simulink model "ASM_AnimationInterface"  (R2024a)
settings: Solver=ode1  StartTime=SIM.tstart.v  StopTime=SIM.tend.v  FixedStep=SIM.StepSize.v  RelTol=1e-3
PostLoadFcn:
  | , if any(exist('dsrtsu_mdlpostloadfcn', 'file') ~= 0), dsrtsu_mdlpostloadfcn('Execute', bdroot); end,
undefined symbols (not defined in the file): a0b2, b98103fe8ad365046cd0, dsmsi, MDL, SIM
libraries: simulink x22, dsmsilib x15, dsmpblib x4, ASM_Environment_lib x1
(part 1 of 7)
settings Model: RTICANMMDATA=struct('GeneralSetupData',struct('modelroot','C:\_GIT\ASM\Demo\Common\Simulation\Models','generalsettings',struct('filesettings',struct('destfolder',struct('Name','RTICANMM_FILES','Check',1),'buildfolder',struct('Name','.','Check',1),'AbsDestfolder',struct('Name','C:\_GIT\ASM\Demo\Common\Simulation\Models\RTICANMM_FILES'),'AbsBuildfolder',struct('Name','C:\_GIT\ASM\Demo\Common\Simulation\Models'))),'options',struct('addpaths',1,'rmpaths',1,'addtrcexclusion',true,'cannavigator',struct('checkmonitoring',0),'show_usrtrc',0,'use_usrtrc',0),'advanced',struct('options',ones(1,100)),'MPSetup',{{}},'RTI',struct('Type','GRT','Ver','','Date',''),'modelname','ASM_AnimationInterface','block','ASM_AnimationInterface'))  RTILINMMDATA=struct('GeneralSetupData',[])  DSRTSU_INTERNAL_RTI_VER=680  DSRTSU_INTERNAL_RTI_TYPE=rti1202  DSRTSU_INTERNAL_MDBS_VER=10  DSRTSU_INTERNAL_RTIFPGA=231  DSMPB_ID_DATA={'213406',struct('BlockId','196758cd-f01c-424e-aa71-f09de9b2c735','SignalIds',{{'6bbc41e1-0e49-4599-bed1-e27503c69a6b','b0969e61-917d-4221-8d62-1269ab223ac8'}}),'213407',struct('BlockId','6fc9ca26-9143-4720-acd9-f350a67d1c14','SignalIds',{{'88eab67c-f0eb-465f-8586-3b7bd00cb24a'}}),'213408',struct('BlockId','3cf7e26e-2ba5-4f6c-9896-28141b6d82c0','SignalIds',{{'8521c402-61b4-4fd4-94cf-d9926b9aa0e5'}}),'213409',struct('BlockId','5820cfdf-8ef4-4d35-adbb-082004934516','SignalIds',{{'6ca39ae5-80bb-46c1-91c4-90194903fd58','bdebb698-3ad2-4907-af9b-3ee7a1752205'}})}  DSRTSU_INTERNAL_RTISTBM_VER=26.1  Creator=RainerF  LastModifiedBy=dSPACE GmbH
settings SolverCC: AlgebraicLoopSolver=TrustRegion
settings DataIOCC: LimitDataPoints=on  SaveFormat=Structure  SignalLoggingSaveFormat=ModelDataLogs  SaveOutput=off  SignalLogging=off  DSMLogging=off  SaveTime=off  ReturnWorkspaceOutputs=off  SignalLoggingName=sigsOut
settings OptimizationCC: BlockReduction=off  BooleanDataType=off  ConditionallyExecuteInputs=off  OptimizeBlockIOStorage=off  BufferReuse=off  ReuseModelBlockBuffer=off  GlobalBufferReuse=off  ExpressionFolding=off  ExpressionDepthLimit=2147483647  LocalBlockOutputs=off  InitFltsAndDblsToZero=on  LifeSpan=inf  OptimizeDataStoreBuffers=off  BusAssignmentInplaceUpdate=off
settings DebuggingCC: SignalInfNanChecking=warning  SaveWithParameterizedLinksMsg=none  SignalResolutionControl=TryResolveAllWithWarning  MultiTaskDSMMsg=warning  MultiTaskCondExecSysMsg=none  CheckMatrixSingularityMsg=warning  FcnCallInpInsideContextMsg=warning  UnconnectedInputMsg=warning  UnconnectedOutputMsg=warning  UnconnectedLineMsg=warning  AllowSymbolicDim=off  StateNameClashWarn=warning  PregeneratedLibrarySubsystemCodeDiagnostic=none  StrictBusMsg=ErrorOnBusTreatedAsVector  NonBusSignalsTreatedAsBus=error  SFUnexpectedBacktrackingDiag=warning  SFNoUnconditionalDefaultTransitionDiag=warning  SFExecutionAtInitializationDiag=none  ArithmeticOperatorsInVariantConditions=warning
settings HardwareCC: ProdBitPerPointer=32  ProdBitPerSizeT=32  ProdBitPerPtrDiffT=32  ProdLargestAtomicFloat=None  ProdWordSize=32  ProdLongLongMode=on  ProdHWDeviceType=Specified  TargetIntDivRoundTo=Zero  TargetEndianess=LittleEndian
settings ModelReferenceCC: EnableRefExpFcnMdlSchedulingChecks=on  PropagateSignalLabelsOutOfModel=off
settings SFSimCC: SimUseLocalCustomCode=off  CustomCodeUndefinedFunction=UseInterfaceOnly
settings RTWCC: Description=dSPACE DS1006 Hardware Platform  RetainRTWFile=on  RTWUseLocalCustomCode=off  GPUComputeCapability=3.5  DLArmComputeVersion=19.05
settings CodeAppCC: StateflowObjectComments=on
settings GRTTargetCC: TargetFcnLib=ansi_tfl_tmw.mat  TargetLangStandard=C89/C90 (ANSI)  CombineOutputUpdateFcns=off  GRTInterface=on
settings ConfigComp: CovMetricSettings=dw  CovSaveCumulativeToWorkspaceVar=on  CovSaveSingleToWorkspaceVar=on  CovExternalEMLEnable=off  CovSFcnEnable=off

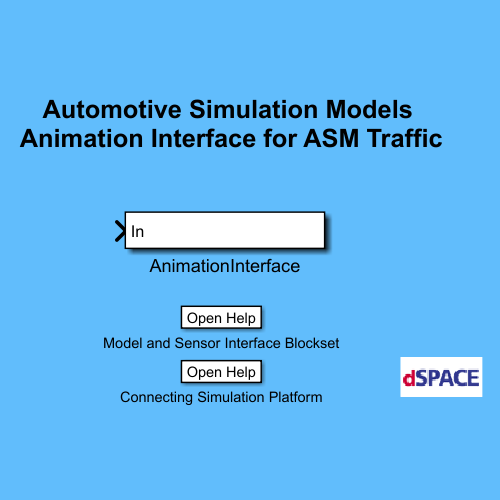
[thumbnail: Simulink's stored preview of the top-level diagram]
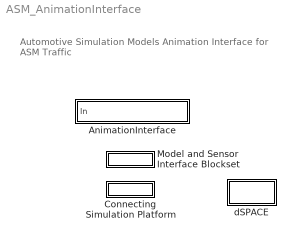
== system ASM_AnimationInterface ==
  note: Automotive Simulation Models
      | Animation Interface for ASM Traffic
  AnimationInterface : Subsystem  Tag=AnimationInterface
  Connecting Simulation Platform : Subsystem
      settings: OpenFcn=dsmsi_help('Help_ConnectingSimulationPlatforms')
      mask Display: disp('Open Help');
  Model and Sensor Interface Blockset : Subsystem
      settings: OpenFcn=dsmsi_help('HELP')
      mask Display: disp('Open Help');
  dSPACE : Subsystem
      mask Display: image(imread('asm_lib_dslogo.tif'));

== system ASM_AnimationInterface/AnimationInterface ==
  note: Animation Interface
  In : Inport
  ANIMATION_INTERFACE : Subsystem
  Bus Selector : BusSelector  OutputSignals=Environment.Animation.Sw_AnimationInterface[0Disabled|1Enabled],Environment.Animation.ManeuverState[]
  DriverAssistance_Animation : BusSelector  OutputSignals=DomainControl.DriverAssistance.Animation  OutputAsBus=on
  Drivetrain_Animation : BusSelector  OutputSignals=Drivetrain.Animation  OutputAsBus=on
  Environment_Animation : BusSelector  OutputSignals=Environment.Animation  OutputAsBus=on
  FcnCall : Subsystem
  Fellow_Doors : Subsystem
  Fellow_Lights : Subsystem
  OpenAnimationInterfaceModel : Subsystem
      settings: OpenFcn=|
      | InterfaceModel = 'ASM_AnimationInterface';
      | 
      | try
      |     open_system(InterfaceModel);                         catch
      |     errordlg(['ERROR opening Animation interface: ',InterfaceModel,'.slx']);
      | end
      mask Display: disp('Open ASM_AnimationInterface')
  Rate Transition{,1..3} (4 alike) : RateTransition  Integrity=off  OutPortSampleTimeOpt=Inherit
  VehicleDynamics_Animation : BusSelector  OutputSignals=VehicleDynamics.Animation  OutputAsBus=on
  Vehicle_Doors : Subsystem
  Vehicle_Lights : Subsystem
  wires:
  In/1 -> Bus Selector/1, DriverAssistance_Animation/1, Drivetrain_Animation/1, Environment_Animation/1, VehicleDynamics_Animation/1
  VehicleDynamics_Animation/1 -> Rate Transition3/1
  DriverAssistance_Animation/1 -> Rate Transition/1
  Environment_Animation/1 -> Rate Transition2/1
  Rate Transition/1 -> ANIMATION_INTERFACE/1(DriverAssistance_Animation)
  Rate Transition1/1 -> ANIMATION_INTERFACE/2(Drivetrain_Animation)
  Drivetrain_Animation/1 -> Rate Transition1/1
  Bus Selector/2 -> FcnCall/1(ManeuverState[])  "<ManeuverState[]>"
  FcnCall/1(FcnCallEvent[]) -> ANIMATION_INTERFACE/Trigger
  Rate Transition3/1 -> Vehicle_Lights/1(VehicleDynamics_Animation), ANIMATION_INTERFACE/3(VehicleDynamics_Animation)
  Fellow_Lights/1(Fellow_Light) -> ANIMATION_INTERFACE/6(Fellow_Lights)
  Vehicle_Lights/1(ASM_Vehicle_Lights) -> ANIMATION_INTERFACE/5(ASM_Vehicle_Lights)
  Rate Transition2/1 -> Fellow_Lights/1(Environment_Animation), Vehicle_Doors/1(Environment_Animation), Fellow_Doors/1(Environment_Animation), Vehicle_Lights/2(Environment_Animation), ANIMATION_INTERFACE/4(Environment_Animation)
  Vehicle_Doors/1(ASM_Vehicle_Doors) -> ANIMATION_INTERFACE/7(ASM_Vehicle_Doors)
  Fellow_Doors/1(Fellow_Doors) -> ANIMATION_INTERFACE/8(Fellow_Doors)
  Bus Selector/1 -> FcnCall/Enable  "<Sw_AnimationInterface[0Disabled|1Enabled]>"

== system ASM_AnimationInterface/Connecting Simulation Platform ==

== system ASM_AnimationInterface/Model and Sensor Interface Blockset ==

== system ASM_AnimationInterface/dSPACE ==

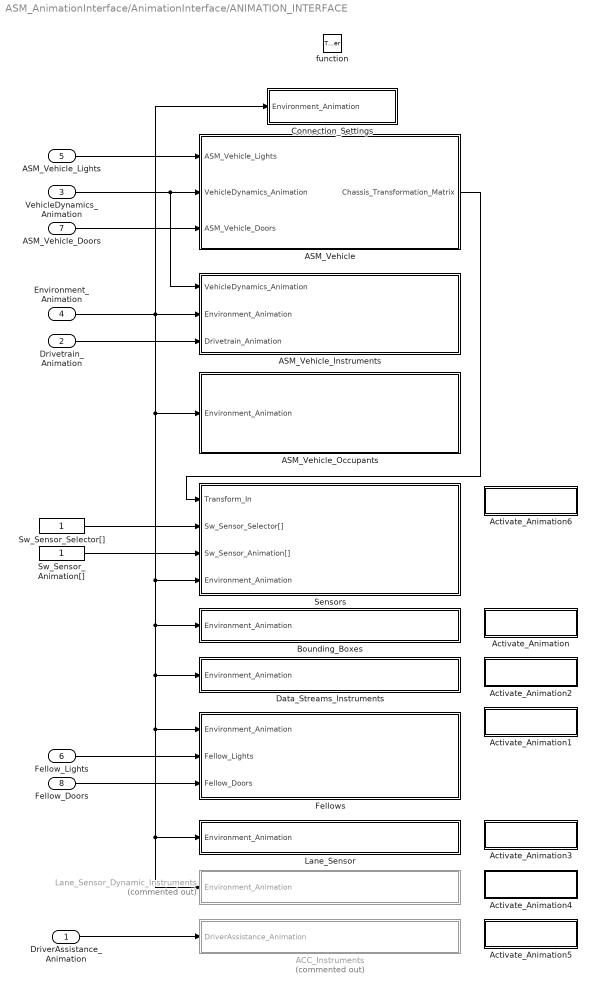
== system ASM_AnimationInterface/AnimationInterface/ANIMATION_INTERFACE ==
  DriverAssistance_Animation : Inport
  Drivetrain_Animation : Inport  Port=2
  VehicleDynamics_Animation : Inport  Port=3
  Environment_Animation : Inport  Port=4
  ASM_Vehicle_Lights : Inport  Port=5
  Fellow_Lights : Inport  Port=6
  ASM_Vehicle_Doors : Inport  Port=7
  Fellow_Doors : Inport  Port=8
  function : TriggerPort  TriggerType=function-call  VariantControl=Variant
  ACC_Instruments : Subsystem  Tag=Animation_ACC_Instruments  Priority=10001  Commented=on
  ASM_Vehicle : Subsystem  Tag=Animation_ASM_Vehicle  Priority=10001
  ASM_Vehicle_Instruments : Subsystem  Tag=Animation_ASM_Vehicle_Instruments  Priority=10001
  ASM_Vehicle_Occupants : Subsystem  Tag=Animation_ASM_Vehicle_Occupants  Priority=10001
  Activate_Animation : Subsystem  mask{ASMVehicle=Uncomment, ASMVehicleInstruments=Uncomment, ASMSensors=Uncomment, BoundigBoxes=Uncomment}
      mask prompts: ASMVehicle "ASM Vehicle"; ASMVehicleInstruments "ASM Vehicle Instruments"; ASMSensors "ASM Sensors"; BoundigBoxes "Bounding Boxes"
      settings: OpenFcn=|
      | subsysTag = 'Animation_Bounding_Boxes';
      | subsys = find_system(get_param(gcb,'Parent'),'SearchDepth','1','IncludeCommented','on','Tag',subsysTag);
      | if ~isempty(subsys)
      |     subsysState = get_param(subsys,'commented');
      |     if strcmp(subsysState,'off')
      |         set_param(subsys{1},'commented','on')
      |     end
      |     if strcmp(subsysState,'on')
      |         set_param(subsys{1},'commented','off')
      |     end
      | else
      |     disp(['Subsystem tagged with ''', subsysTag, ''' could not be found. The button is without action.'])
      | end
      mask TypeOptions ASMVehicle: Comment out | Uncomment
      mask Callback ASMVehicle: asm_vehicle_comment(gcb)
      mask TypeOptions ASMVehicleInstruments: Comment out | Uncomment
      mask TypeOptions ASMSensors: Comment out | Uncomment
      mask Callback ASMSensors:
      | subsys = find_system(get_param(gcb,'Parent'),'SearchDepth','1','IncludeCommented','on','Tag','ASM_Sensors');
      | if ~isempty(subsys)
      |     button_state = get_param(gcb,'ASMSensors');
      |     subsys_state = get_param(subsys,'commented');
      |     if strcmp(button_state,'Comment out') && strcmp(subsys_state,'off')
      |         set_param(subsys{1},'commented','on')
      |     end
      |     if strcmp(button_state,'Uncomment') && strcmp(subsys_state,'on')
      |         set_param(subsys{1},'commented','off')
      |     end
      | end
      mask TypeOptions BoundigBoxes: Comment out | Uncomment
      mask Display: disp('double click to\n activate/deactivate')
  Activate_Animation1 : Subsystem  mask{ASMVehicle=Uncomment, ASMVehicleInstruments=Uncomment, ASMSensors=Uncomment, BoundigBoxes=Uncomment}
      mask prompts: ASMVehicle "ASM Vehicle"; ASMVehicleInstruments "ASM Vehicle Instruments"; ASMSensors "ASM Sensors"; BoundigBoxes "Bounding Boxes"
      settings: OpenFcn=|
      | subsysTag = 'Animation_Fellows';
      | subsys = find_system(get_param(gcb,'Parent'),'SearchDepth','1','IncludeCommented','on','Tag',subsysTag);
      | if ~isempty(subsys)
      |     subsysState = get_param(subsys,'commented');
      |     if strcmp(subsysState,'off')
      |         set_param(subsys{1},'commented','on')
      |     end
      |     if strcmp(subsysState,'on')
      |         set_param(subsys{1},'commented','off')
      |     end
      | else
      |     disp(['Subsystem tagged with ''', subsysTag, ''' could not be found. The button is without action.'])
      | end
      mask TypeOptions ASMVehicle: Comment out | Uncomment
      mask Callback ASMVehicle: asm_vehicle_comment(gcb)
      mask TypeOptions ASMVehicleInstruments: Comment out | Uncomment
      mask TypeOptions ASMSensors: Comment out | Uncomment
      mask Callback ASMSensors:
      | subsys = find_system(get_param(gcb,'Parent'),'SearchDepth','1','IncludeCommented','on','Tag','ASM_Sensors');
      | if ~isempty(subsys)
      |     button_state = get_param(gcb,'ASMSensors');
      |     subsys_state = get_param(subsys,'commented');
      |     if strcmp(button_state,'Comment out') && strcmp(subsys_state,'off')
      |         set_param(subsys{1},'commented','on')
      |     end
      |     if strcmp(button_state,'Uncomment') && strcmp(subsys_state,'on')
      |         set_param(subsys{1},'commented','off')
      |     end
      | end
      mask TypeOptions BoundigBoxes: Comment out | Uncomment
      mask Display: disp('double click to\n activate/deactivate')
  Activate_Animation2 : Subsystem  mask{ASMVehicle=Uncomment, ASMVehicleInstruments=Uncomment, ASMSensors=Uncomment, BoundigBoxes=Uncomment}
      mask prompts: ASMVehicle "ASM Vehicle"; ASMVehicleInstruments "ASM Vehicle Instruments"; ASMSensors "ASM Sensors"; BoundigBoxes "Bounding Boxes"
      settings: OpenFcn=|
      | subsysTag = 'Animation_Data_Streams_Instruments';
      | subsys = find_system(get_param(gcb,'Parent'),'SearchDepth','1','IncludeCommented','on','Tag',subsysTag);
      | if ~isempty(subsys)
      |     subsysState = get_param(subsys,'commented');
      |     if strcmp(subsysState,'off')
      |         set_param(subsys{1},'commented','on')
      |     end
      |     if strcmp(subsysState,'on')
      |         set_param(subsys{1},'commented','off')
      |     end
      | else
      |     disp(['Subsystem tagged with ''', subsysTag, ''' could not be found. The button is without action.'])
      | end
      mask TypeOptions ASMVehicle: Comment out | Uncomment
      mask Callback ASMVehicle: asm_vehicle_comment(gcb)
      mask TypeOptions ASMVehicleInstruments: Comment out | Uncomment
      mask TypeOptions ASMSensors: Comment out | Uncomment
      mask Callback ASMSensors:
      | subsys = find_system(get_param(gcb,'Parent'),'SearchDepth','1','IncludeCommented','on','Tag','ASM_Sensors');
      | if ~isempty(subsys)
      |     button_state = get_param(gcb,'ASMSensors');
      |     subsys_state = get_param(subsys,'commented');
      |     if strcmp(button_state,'Comment out') && strcmp(subsys_state,'off')
      |         set_param(subsys{1},'commented','on')
      |     end
      |     if strcmp(button_state,'Uncomment') && strcmp(subsys_state,'on')
      |         set_param(subsys{1},'commented','off')
      |     end
      | end
      mask TypeOptions BoundigBoxes: Comment out | Uncomment
      mask Display: disp('double click to\n activate/deactivate')
  Activate_Animation3 : Subsystem  mask{ASMVehicle=Uncomment, ASMVehicleInstruments=Uncomment, ASMSensors=Uncomment, BoundigBoxes=Uncomment}
      mask prompts: ASMVehicle "ASM Vehicle"; ASMVehicleInstruments "ASM Vehicle Instruments"; ASMSensors "ASM Sensors"; BoundigBoxes "Bounding Boxes"
      settings: OpenFcn=|
      | subsysTag = 'Animation_Lane_Sensor';
      | subsys = find_system(get_param(gcb,'Parent'),'SearchDepth','1','IncludeCommented','on','Tag',subsysTag);
      | if ~isempty(subsys)
      |     subsysState = get_param(subsys,'commented');
      |     if strcmp(subsysState,'off')
      |         set_param(subsys{1},'commented','on')
      |     end
      |     if strcmp(subsysState,'on')
      |         set_param(subsys{1},'commented','off')
      |     end
      | else
      |     disp(['Subsystem tagged with ''', subsysTag, ''' could not be found. The button is without action.'])
      | end
      mask TypeOptions ASMVehicle: Comment out | Uncomment
      mask Callback ASMVehicle: asm_vehicle_comment(gcb)
      mask TypeOptions ASMVehicleInstruments: Comment out | Uncomment
      mask TypeOptions ASMSensors: Comment out | Uncomment
      mask Callback ASMSensors:
      | subsys = find_system(get_param(gcb,'Parent'),'SearchDepth','1','IncludeCommented','on','Tag','ASM_Sensors');
      | if ~isempty(subsys)
      |     button_state = get_param(gcb,'ASMSensors');
      |     subsys_state = get_param(subsys,'commented');
      |     if strcmp(button_state,'Comment out') && strcmp(subsys_state,'off')
      |         set_param(subsys{1},'commented','on')
      |     end
      |     if strcmp(button_state,'Uncomment') && strcmp(subsys_state,'on')
      |         set_param(subsys{1},'commented','off')
      |     end
      | end
      mask TypeOptions BoundigBoxes: Comment out | Uncomment
      mask Display: disp('double click to\n activate/deactivate')
  Activate_Animation4 : Subsystem  mask{ASMVehicle=Uncomment, ASMVehicleInstruments=Uncomment, ASMSensors=Uncomment, BoundigBoxes=Uncomment}
      mask prompts: ASMVehicle "ASM Vehicle"; ASMVehicleInstruments "ASM Vehicle Instruments"; ASMSensors "ASM Sensors"; BoundigBoxes "Bounding Boxes"
      settings: OpenFcn=|
      | subsysTag = 'Animation_Lane_Sensor_Dynamic_Instruments';
      | subsys = find_system(get_param(gcb,'Parent'),'SearchDepth','1','IncludeCommented','on','Tag',subsysTag);
      | if ~isempty(subsys)
      |     subsysState = get_param(subsys,'commented');
      |     if strcmp(subsysState,'off')
      |         set_param(subsys{1},'commented','on')
      |     end
      |     if strcmp(subsysState,'on')
      |         set_param(subsys{1},'commented','off')
      |     end
      | else
      |     disp(['Subsystem tagged with ''', subsysTag, ''' could not be found. The button is without action.'])
      | end
      mask TypeOptions ASMVehicle: Comment out | Uncomment
      mask Callback ASMVehicle: asm_vehicle_comment(gcb)
      mask TypeOptions ASMVehicleInstruments: Comment out | Uncomment
      mask TypeOptions ASMSensors: Comment out | Uncomment
      mask Callback ASMSensors:
      | subsys = find_system(get_param(gcb,'Parent'),'SearchDepth','1','IncludeCommented','on','Tag','ASM_Sensors');
      | if ~isempty(subsys)
      |     button_state = get_param(gcb,'ASMSensors');
      |     subsys_state = get_param(subsys,'commented');
      |     if strcmp(button_state,'Comment out') && strcmp(subsys_state,'off')
      |         set_param(subsys{1},'commented','on')
      |     end
      |     if strcmp(button_state,'Uncomment') && strcmp(subsys_state,'on')
      |         set_param(subsys{1},'commented','off')
      |     end
      | end
      mask TypeOptions BoundigBoxes: Comment out | Uncomment
      mask Display: disp('double click to\n activate/deactivate')
  Activate_Animation5 : Subsystem  mask{ASMVehicle=Uncomment, ASMVehicleInstruments=Uncomment, ASMSensors=Uncomment, BoundigBoxes=Uncomment}
      mask prompts: ASMVehicle "ASM Vehicle"; ASMVehicleInstruments "ASM Vehicle Instruments"; ASMSensors "ASM Sensors"; BoundigBoxes "Bounding Boxes"
      settings: OpenFcn=|
      | subsysTag = 'Animation_ACC_Instruments';
      | subsys = find_system(get_param(gcb,'Parent'),'SearchDepth','1','IncludeCommented','on','Tag',subsysTag);
      | if ~isempty(subsys)
      |     subsysState = get_param(subsys,'commented');
      |     if strcmp(subsysState,'off')
      |         set_param(subsys{1},'commented','on')
      |     end
      |     if strcmp(subsysState,'on')
      |         set_param(subsys{1},'commented','off')
      |     end
      | else
      |     disp(['Subsystem tagged with ''', subsysTag, ''' could not be found. The button is without action.'])
      | end
      mask TypeOptions ASMVehicle: Comment out | Uncomment
      mask Callback ASMVehicle: asm_vehicle_comment(gcb)
      mask TypeOptions ASMVehicleInstruments: Comment out | Uncomment
      mask TypeOptions ASMSensors: Comment out | Uncomment
      mask Callback ASMSensors:
      | subsys = find_system(get_param(gcb,'Parent'),'SearchDepth','1','IncludeCommented','on','Tag','ASM_Sensors');
      | if ~isempty(subsys)
      |     button_state = get_param(gcb,'ASMSensors');
      |     subsys_state = get_param(subsys,'commented');
      |     if strcmp(button_state,'Comment out') && strcmp(subsys_state,'off')
      |         set_param(subsys{1},'commented','on')
      |     end
      |     if strcmp(button_state,'Uncomment') && strcmp(subsys_state,'on')
      |         set_param(subsys{1},'commented','off')
      |     end
      | end
      mask TypeOptions BoundigBoxes: Comment out | Uncomment
      mask Display: disp('double click to\n activate/deactivate')
  Activate_Animation6 : Subsystem  mask{ASMVehicle=Uncomment, ASMVehicleInstruments=Uncomment, ASMSensors=Uncomment, BoundigBoxes=Uncomment}
      mask prompts: ASMVehicle "ASM Vehicle"; ASMVehicleInstruments "ASM Vehicle Instruments"; ASMSensors "ASM Sensors"; BoundigBoxes "Bounding Boxes"
      settings: OpenFcn=|
      | subsysTag = 'Animation_Sensors';
      | subsys = find_system(get_param(gcb,'Parent'),'SearchDepth','1','IncludeCommented','on','Tag',subsysTag);
      | if ~isempty(subsys)
      |     subsysState = get_param(subsys,'commented');
      |     if strcmp(subsysState,'off')
      |         set_param(subsys{1},'commented','on')
      |     end
      |     if strcmp(subsysState,'on')
      |         set_param(subsys{1},'commented','off')
      |     end
      | else
      |     disp(['Subsystem tagged with ''', subsysTag, ''' could not be found. The button is without action.'])
      | end
      mask TypeOptions ASMVehicle: Comment out | Uncomment
      mask Callback ASMVehicle: asm_vehicle_comment(gcb)
      mask TypeOptions ASMVehicleInstruments: Comment out | Uncomment
      mask TypeOptions ASMSensors: Comment out | Uncomment
      mask Callback ASMSensors:
      | subsys = find_system(get_param(gcb,'Parent'),'SearchDepth','1','IncludeCommented','on','Tag','ASM_Sensors');
      | if ~isempty(subsys)
      |     button_state = get_param(gcb,'ASMSensors');
      |     subsys_state = get_param(subsys,'commented');
      |     if strcmp(button_state,'Comment out') && strcmp(subsys_state,'off')
      |         set_param(subsys{1},'commented','on')
      |     end
      |     if strcmp(button_state,'Uncomment') && strcmp(subsys_state,'on')
      |         set_param(subsys{1},'commented','off')
      |     end
      | end
      mask TypeOptions BoundigBoxes: Comment out | Uncomment
      mask Display: disp('double click to\n activate/deactivate')
  Bounding_Boxes : Subsystem  Tag=Animation_Bounding_Boxes  Priority=10001
  Connection_Settings : Subsystem  Tag=AnimationInterface_Connection_Settings  Priority=10009  mask(Connection_Settings){CommunicationMethod=Communication Service, Sw_Mode=0, ModelStepSize=SIM.StepSize.v, NumSamples=SIM.NumSamplesAnimation.v, MaxMessageSize=65507}
      mask prompts: CommunicationMethod "Communication method"; Sw_Mode "Simulation mode [0SIL|1HIL]"; ModelStepSize "Step size of the model [s]"; NumSamples "Time steps between two sent messages []"; MaxMessageSize "Maximum message size [bytes]"
      mask help: Specifies the communication method for transferring the collected simulation data to a consuming application.
      mask TypeOptions CommunicationMethod: Ethernet TCP | Communication Service
      mask Callback CommunicationMethod:
      | CommunicationMethod = Simulink.Mask.get(gcb).getParameter('CommunicationMethod'); % Ethernet TCP; Communication Service
      | 
      |     % Get Mask Dialogs & Controls
      |     EthernetTCPDescription      = Simulink.Mask.get(gcb).getDialogControl('EthernetTCPDescription');
      |     COMServiceDescription       = Simulink.Mask.get(gcb).getDialogControl('COMServiceDescription');
      |     AdvancedSettingsContainer   = Simulink.Mask.get(gcb).getDialogControl('AdvancedSettings');
      | 
      |     % Get Ethernet TCP Parameter
      |     Sw_Mode                     = Simulink.Mask.get(gcb).getParameter('Sw_Mode'); % SIL or HIL
      | 
      |     % Get Communication Service Parameter
      |     ModelStepSize               = Simulink.Mask.get(gcb).getParameter('ModelStepSize');
      |     NumSamples                  = Simulink.Mask.get(gcb).getParameter('NumSamples');
      |     MaxMessageSize              = Simulink.Mask.get(gcb).getParameter('MaxMessageSize');
      | 
      |     % Get blocks inside the masked subsystem
      |     SwCommunicationMethod           = [gcb,'/Sw_CommunicationMethod[0TCP|1ComService]'];     % Constant block for switching the Communication Method
      |     SubSysEthernetTCP               = [gcb,'/Ethernet_TCP'];
      |     SubSysCommunicationService      = [gcb,'/Communication_Service'];
      | 
      |     if strcmp(CommunicationMethod.Value, 'Ethernet TCP')
      |         set_param(SwCommunicationMethod, 'Value','0');
      | 
      |         % Set Ethernet TCP Visibilities
      |         Sw_Mode.Visible                 = 'on';
      |         EthernetTCPDescription.Visible  = 'on';
      |         set_param(SubSysEthernetTCP,'commented','off')
      | 
      |         % Set Communication Service Visibilities
      |         AdvancedSettingsContainer.Visible   = 'off';
      |         ModelStepSize.Visible               = 'off';
      |         NumSamples.Visible                  = 'off';
      |         MaxMessageSize.Visible              = 'off';
      |         COMServiceDescription.Visible       = 'off';
      |         set_param(SubSysCommunicationService,'commented','on')
      |     elseif strcmp(CommunicationMethod.Value, 'Communication Service')
      |         set_param(SwCommunicationMethod, 'Value','1');
      | 
      |         % Set Ethernet TCP Visibilities
      |         Sw_Mode.Visible                 = 'off';
      |         EthernetTCPDescription.Visible  = 'off';
      |         set_param(SubSysEthernetTCP,'commented','on')
      | 
      |         % Set Communication Service Visibilities
      |         AdvancedSettingsContainer.Visible   = 'on';
      |         ModelStepSize.Visible               = 'on';
      |         NumSamples.Visible                  = 'on';
      |         MaxMessageSize.Visible              = 'on';
      |         COMServiceDescription.Visible       = 'on';
      |         set_param(SubSysCommunicationService,'commented','off')
      |     end
      mask Callback Sw_Mode:
      | simMode     = get_param(gcb, 'Sw_Mode');
      |     subsysSIL   = [gcb,'/Ethernet_TCP/SIL'];
      |     subsysHIL   = [gcb,'/Ethernet_TCP/HIL'];
      | 
      |     if strcmp(simMode,'0') % SIL
      |         if strcmp(get_param(subsysSIL,'commented'),'on')
      |             set_param(subsysSIL,'commented','off')
      |         end
      |         if strcmp(get_param(subsysHIL,'commented'),'off')
      |             set_param(subsysHIL,'commented','on')
      |         end
      |     elseif strcmp(simMode,'1') % HIL
      |         if strcmp(get_param(subsysHIL,'commented'),'on')
      |             set_param(subsysHIL,'commented','off')
      |         end
      |         if strcmp(get_param(subsysSIL,'commented'),'off')
      |             set_param(subsysSIL,'commented','on')
      |         end
      |     else
      |         disp(['Invalid parameter value of ''', gcb, '''. Allowed values are 0 and 1'])
      |     end
      mask TypeOptions ModelStepSize: Communication_Service/dsmsi_communication_service_BL1/ModelStepSize
      mask TypeOptions NumSamples: Communication_Service/dsmsi_communication_service_BL1/NumSamples
      mask TypeOptions MaxMessageSize: Communication_Service/dsmsi_communication_service_BL1/MaxMessageSize
      mask DialogControl EthernetTCPDescription Prompt: The Ethernet TCP connection supports the following Platforms: <br> Simulation Mode <b>SIL</b>: Simulink, VEOS <br> Simulation Mode <b>HIL</b>: SCALEXIO
      mask DialogControl COMServiceDescription Prompt: For supported platforms, please refer to the help of the "ASM_COMMUNICATION_SERVICE" block.
      mask DialogControl Settings Prompt: Settings
      mask DialogControl AdvancedSettings Prompt: Advanced settings
      mask Display: disp('Configure\n Connection Settings')
  Data_Streams_Instruments : Subsystem  Tag=Animation_Data_Streams_Instruments  Priority=10001
  Fellows : Subsystem  Tag=Animation_Fellows  Priority=10001
  Lane_Sensor : Subsystem  Tag=Animation_Lane_Sensor  Priority=10001
  Lane_Sensor_Dynamic_Instruments : Subsystem  Tag=Animation_Lane_Sensor_Dynamic_Instruments  Priority=10001  Commented=on
  Sensors : Subsystem  Tag=Animation_Sensors  Priority=10001
  Sw_Sensor_Animation[] : Constant
      settings: AttributesFormatString=1_Object3D\n2_Object2D\n3_TrafficSign\n4_LineSensor_Road_Lanes\n5_LineSensor_Road_Shape_Lines\n6_LineSensor_Road_Shape_ContObj\n7_LineSensor_Junction_Borders\n8_LineSensor_Junction_Shape_Lines\n9_LineSensor_Junction_Shape_ContObj\n10_Object3D_RadarEffects\n11_Object3D_CustomPoints
  Sw_Sensor_Selector[] : Constant
  wires:
  DriverAssistance_Animation/1 -> ACC_Instruments/1(DriverAssistance_Animation)
  VehicleDynamics_Animation/1 -> ASM_Vehicle_Instruments/1(VehicleDynamics_Animation), ASM_Vehicle/2(VehicleDynamics_Animation)
  ASM_Vehicle/1(Chassis_Transformation_Matrix) -> Sensors/1(Transform_In)
  Drivetrain_Animation/1 -> ASM_Vehicle_Instruments/3(Drivetrain_Animation)
  Sw_Sensor_Animation[]/1 -> Sensors/3(Sw_Sensor_Animation[])
  Sw_Sensor_Selector[]/1 -> Sensors/2(Sw_Sensor_Selector[])
  Fellow_Lights/1 -> Fellows/2(Fellow_Lights)
  ASM_Vehicle_Lights/1 -> ASM_Vehicle/1(ASM_Vehicle_Lights)
  ASM_Vehicle_Doors/1 -> ASM_Vehicle/3(ASM_Vehicle_Doors)
  Fellow_Doors/1 -> Fellows/3(Fellow_Doors)
  Environment_Animation/1 -> ASM_Vehicle_Occupants/1(Environment_Animation), Sensors/4(Environment_Animation), Bounding_Boxes/1(Environment_Animation), Data_Streams_Instruments/1(Environment_Animation), Fellows/1(Environment_Animation), Lane_Sensor/1(Environment_Animation), Lane_Sensor_Dynamic_Instruments/1(Environment_Animation), Connection_Settings/1(Environment_Animation), ASM_Vehicle_Instruments/2(Environment_Animation)

== system ASM_AnimationInterface/AnimationInterface/FcnCall ==
  ManeuverState[] : Inport
  Enable1 : EnablePort
  Disable : Constant  Value=0  OutDataTypeStr=Inherit: Inherit via back propagation
  Enable : Constant  OutDataTypeStr=Inherit: Inherit via back propagation
  External_Samples : Subsystem  TreatAsAtomicUnit=on  SystemSampleTime=SIM.StepSize.v
      settings: AttributesFormatString=Ts=%<SystemSampleTime>
  MANEUVER_FCN_CALL_GENERATOR : ASM_Environment_lib/Environment/Maneuver/MANEUVER_FCN_CALL_GENERATOR  NumSamples=SIM.NumSamplesAnimation.v  ASMProperties=struct('Name','MANEUVER_FCN_CALL_GENERATOR','Version','3.0','Library','ASM_Environment_lib')  ASMInstanceName=maneuver_fcn_call_generator  ASMInstanceID=1
  Samples_Ext[] : Constant  OutDataTypeStr=Inherit: Inherit via back propagation
  Switch : Switch  Criteria=u2 ~= 0  SaturateOnIntegerOverflow=off  InputSameDT=off
  Switch1 : Switch  Criteria=u2 ~= 0  SaturateOnIntegerOverflow=off  InputSameDT=off
  Valid_Samples : simulink/Logic and Bit Operations/Compare To Zero  relop=>  OutDataTypeStr=boolean
  FcnCallEvent[] : Outport
  wires:
  Disable/1 -> Switch1/3
  MANEUVER_FCN_CALL_GENERATOR/1 -> FcnCallEvent[]/1
  ManeuverState[]/1 -> MANEUVER_FCN_CALL_GENERATOR/1
  Enable/1 -> Switch1/1
  Samples_Ext[]/1 -> Switch/3
  Switch1/1 -> MANEUVER_FCN_CALL_GENERATOR/2
  Switch/1 -> MANEUVER_FCN_CALL_GENERATOR/3
  Valid_Samples/1 -> Switch/2, Switch1/2
  External_Samples/1(num_Samples[]) -> Switch/1, Valid_Samples/1

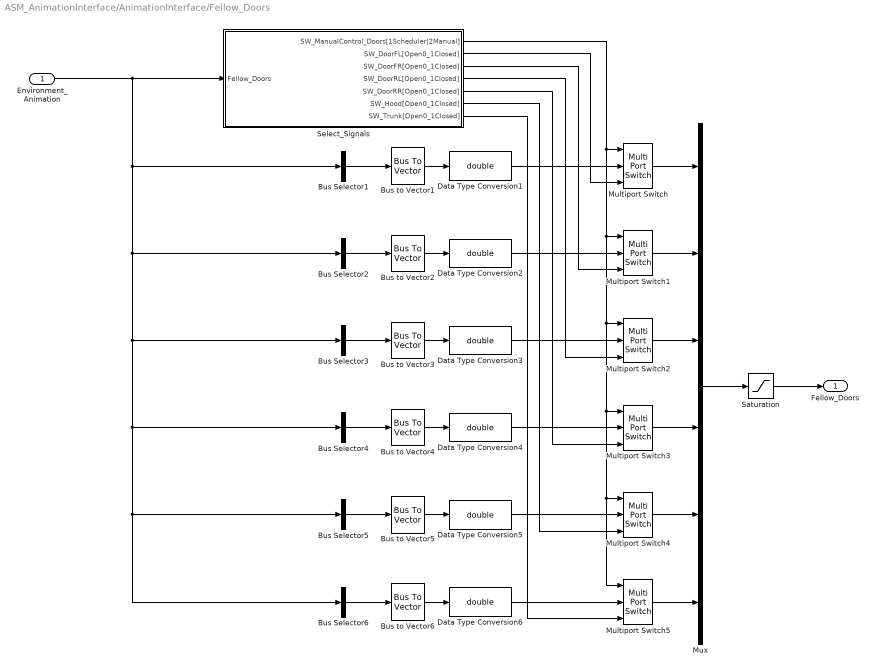
== system ASM_AnimationInterface/AnimationInterface/Fellow_Doors ==
  Environment_Animation : Inport
  Bus Selector1 : BusSelector  OutputSignals=UserSignals_Customized.Fellow1_DoorFL,UserSignals_Customized.Fellow2_DoorFL,UserSignals_Customized.Fellow3_DoorFL,UserSignals_Customized.Fellow4_DoorFL,UserSignals_Customized.Fellow5_DoorFL,UserSignals_Customized.Fellow6_DoorFL,UserSignals_Customized.Fellow7_DoorFL,UserSignals_Customized.Fellow8_DoorFL,UserSignals_Customized.Fellow9_DoorFL,UserSignals_Customized.Fellow10_DoorFL,UserSignals_Customized.Fellow11_DoorFL,UserSignals_Customized.Fellow12_DoorFL,UserSignals_Customized.Fellow13_DoorFL,UserSignals_Customized.Fellow14_DoorFL,UserSignals_Customized.Fellow15_DoorFL,UserSignals_Customized.Fellow16_DoorFL,UserSignals_Customized.Fellow17_DoorFL,UserSignals_Customized.Fellow18_DoorFL,UserSignals_Customized.Fellow19_DoorFL,UserSignals_Customized.Fellow20_DoorFL,UserSignals_Customized.Fellow21_DoorFL,UserSignals_Customized.Fellow22_DoorFL,UserSignals_Customized.Fellow23_DoorFL,UserSignals_Customized.Fellow24_DoorFL,UserSignals_Customized.Fellow25_DoorFL,UserSignals_Customized.Fellow26_DoorFL,UserSignals_Customized.Fellow27_DoorFL,UserSignals_Customized.Fellow28_DoorFL,UserSignals_Customized.Fellow29_DoorFL,UserSignals_Customized.Fellow30_DoorFL  OutputAsBus=on
  Bus Selector2 : BusSelector  OutputSignals=UserSignals_Customized.Fellow1_DoorFR,UserSignals_Customized.Fellow2_DoorFR,UserSignals_Customized.Fellow3_DoorFR,UserSignals_Customized.Fellow4_DoorFR,UserSignals_Customized.Fellow5_DoorFR,UserSignals_Customized.Fellow6_DoorFR,UserSignals_Customized.Fellow7_DoorFR,UserSignals_Customized.Fellow8_DoorFR,UserSignals_Customized.Fellow9_DoorFR,UserSignals_Customized.Fellow10_DoorFR,UserSignals_Customized.Fellow11_DoorFR,UserSignals_Customized.Fellow12_DoorFR,UserSignals_Customized.Fellow13_DoorFR,UserSignals_Customized.Fellow14_DoorFR,UserSignals_Customized.Fellow15_DoorFR,UserSignals_Customized.Fellow16_DoorFR,UserSignals_Customized.Fellow17_DoorFR,UserSignals_Customized.Fellow18_DoorFR,UserSignals_Customized.Fellow19_DoorFR,UserSignals_Customized.Fellow20_DoorFR,UserSignals_Customized.Fellow21_DoorFR,UserSignals_Customized.Fellow22_DoorFR,UserSignals_Customized.Fellow23_DoorFR,UserSignals_Customized.Fellow24_DoorFR,UserSignals_Customized.Fellow25_DoorFR,UserSignals_Customized.Fellow26_DoorFR,UserSignals_Customized.Fellow27_DoorFR,UserSignals_Customized.Fellow28_DoorFR,UserSignals_Customized.Fellow29_DoorFR,UserSignals_Customized.Fellow30_DoorFR  OutputAsBus=on
  Bus Selector3 : BusSelector  OutputSignals=UserSignals_Customized.Fellow1_DoorRL,UserSignals_Customized.Fellow2_DoorRL,UserSignals_Customized.Fellow3_DoorRL,UserSignals_Customized.Fellow4_DoorRL,UserSignals_Customized.Fellow5_DoorRL,UserSignals_Customized.Fellow6_DoorRL,UserSignals_Customized.Fellow7_DoorRL,UserSignals_Customized.Fellow8_DoorRL,UserSignals_Customized.Fellow9_DoorRL,UserSignals_Customized.Fellow10_DoorRL,UserSignals_Customized.Fellow11_DoorRL,UserSignals_Customized.Fellow12_DoorRL,UserSignals_Customized.Fellow13_DoorRL,UserSignals_Customized.Fellow14_DoorRL,UserSignals_Customized.Fellow15_DoorRL,UserSignals_Customized.Fellow16_DoorRL,UserSignals_Customized.Fellow17_DoorRL,UserSignals_Customized.Fellow18_DoorRL,UserSignals_Customized.Fellow19_DoorRL,UserSignals_Customized.Fellow20_DoorRL,UserSignals_Customized.Fellow21_DoorRL,UserSignals_Customized.Fellow22_DoorRL,UserSignals_Customized.Fellow23_DoorRL,UserSignals_Customized.Fellow24_DoorRL,UserSignals_Customized.Fellow25_DoorRL,UserSignals_Customized.Fellow26_DoorRL,UserSignals_Customized.Fellow27_DoorRL,UserSignals_Customized.Fellow28_DoorRL,UserSignals_Customized.Fellow29_DoorRL,UserSignals_Customized.Fellow30_DoorRL  OutputAsBus=on
  Bus Selector4 : BusSelector  OutputSignals=UserSignals_Customized.Fellow1_DoorRR,UserSignals_Customized.Fellow2_DoorRR,UserSignals_Customized.Fellow3_DoorRR,UserSignals_Customized.Fellow4_DoorRR,UserSignals_Customized.Fellow5_DoorRR,UserSignals_Customized.Fellow6_DoorRR,UserSignals_Customized.Fellow7_DoorRR,UserSignals_Customized.Fellow8_DoorRR,UserSignals_Customized.Fellow9_DoorRR,UserSignals_Customized.Fellow10_DoorRR,UserSignals_Customized.Fellow11_DoorRR,UserSignals_Customized.Fellow12_DoorRR,UserSignals_Customized.Fellow13_DoorRR,UserSignals_Customized.Fellow14_DoorRR,UserSignals_Customized.Fellow15_DoorRR,UserSignals_Customized.Fellow16_DoorRR,UserSignals_Customized.Fellow17_DoorRR,UserSignals_Customized.Fellow18_DoorRR,UserSignals_Customized.Fellow19_DoorRR,UserSignals_Customized.Fellow20_DoorRR,UserSignals_Customized.Fellow21_DoorRR,UserSignals_Customized.Fellow22_DoorRR,UserSignals_Customized.Fellow23_DoorRR,UserSignals_Customized.Fellow24_DoorRR,UserSignals_Customized.Fellow25_DoorRR,UserSignals_Customized.Fellow26_DoorRR,UserSignals_Customized.Fellow27_DoorRR,UserSignals_Customized.Fellow28_DoorRR,UserSignals_Customized.Fellow29_DoorRR,UserSignals_Customized.Fellow30_DoorRR  OutputAsBus=on
  Bus Selector5 : BusSelector  OutputSignals=UserSignals_Customized.Fellow1_Hood,UserSignals_Customized.Fellow2_Hood,UserSignals_Customized.Fellow3_Hood,UserSignals_Customized.Fellow4_Hood,UserSignals_Customized.Fellow5_Hood,UserSignals_Customized.Fellow6_Hood,UserSignals_Customized.Fellow7_Hood,UserSignals_Customized.Fellow8_Hood,UserSignals_Customized.Fellow9_Hood,UserSignals_Customized.Fellow10_Hood,UserSignals_Customized.Fellow11_Hood,UserSignals_Customized.Fellow12_Hood,UserSignals_Customized.Fellow13_Hood,UserSignals_Customized.Fellow14_Hood,UserSignals_Customized.Fellow15_Hood,UserSignals_Customized.Fellow16_Hood,UserSignals_Customized.Fellow17_Hood,UserSignals_Customized.Fellow18_Hood,UserSignals_Customized.Fellow19_Hood,UserSignals_Customized.Fellow20_Hood,UserSignals_Customized.Fellow21_Hood,UserSignals_Customized.Fellow22_Hood,UserSignals_Customized.Fellow23_Hood,UserSignals_Customized.Fellow24_Hood,UserSignals_Customized.Fellow25_Hood,UserSignals_Customized.Fellow26_Hood,UserSignals_Customized.Fellow27_Hood,UserSignals_Customized.Fellow28_Hood,UserSignals_Customized.Fellow29_Hood,UserSignals_Customized.Fellow30_Hood  OutputAsBus=on
  Bus Selector6 : BusSelector  OutputSignals=UserSignals_Customized.Fellow1_Trunk,UserSignals_Customized.Fellow2_Trunk,UserSignals_Customized.Fellow3_Trunk,UserSignals_Customized.Fellow4_Trunk,UserSignals_Customized.Fellow5_Trunk,UserSignals_Customized.Fellow6_Trunk,UserSignals_Customized.Fellow7_Trunk,UserSignals_Customized.Fellow8_Trunk,UserSignals_Customized.Fellow9_Trunk,UserSignals_Customized.Fellow10_Trunk,UserSignals_Customized.Fellow11_Trunk,UserSignals_Customized.Fellow12_Trunk,UserSignals_Customized.Fellow13_Trunk,UserSignals_Customized.Fellow14_Trunk,UserSignals_Customized.Fellow15_Trunk,UserSignals_Customized.Fellow16_Trunk,UserSignals_Customized.Fellow17_Trunk,UserSignals_Customized.Fellow18_Trunk,UserSignals_Customized.Fellow19_Trunk,UserSignals_Customized.Fellow20_Trunk,UserSignals_Customized.Fellow21_Trunk,UserSignals_Customized.Fellow22_Trunk,UserSignals_Customized.Fellow23_Trunk,UserSignals_Customized.Fellow24_Trunk,UserSignals_Customized.Fellow25_Trunk,UserSignals_Customized.Fellow26_Trunk,UserSignals_Customized.Fellow27_Trunk,UserSignals_Customized.Fellow28_Trunk,UserSignals_Customized.Fellow29_Trunk,UserSignals_Customized.Fellow30_Trunk  OutputAsBus=on
  Bus to Vector{1..6} (6 alike) : BusToVector
  Data Type Conversion{1..6} (6 alike) : DataTypeConversion  OutDataTypeStr=double  SaturateOnIntegerOverflow=off  RndMeth=Floor
  Multiport Switch : MultiPortSwitch  Inputs=2  OutMin=30  OutMax=30  OutDataTypeStr=double  SaturateOnIntegerOverflow=off
  Multiport Switch{1..5} (5 alike) : MultiPortSwitch  Inputs=2  SaturateOnIntegerOverflow=off  InputSameDT=off
  Mux : Mux  Inputs=6
  Saturation : Saturate  UpperLimit=1  LowerLimit=0
  Select_Signals : Subsystem
  Fellow_Doors : Outport  VectorParamsAs1DForOutWhenUnconnected=off
  wires:
  Select_Signals/1(SW_ManualControl_Doors[1Scheduler|2Manual]) -> Multiport Switch5/1, Multiport Switch4/1, Multiport Switch3/1, Multiport Switch2/1, Multiport Switch1/1, Multiport Switch/1
  Select_Signals/2(SW_DoorFL[Open0_1Closed]) -> Multiport Switch/3
  Bus Selector1/1 -> Bus to Vector1/1
  Bus to Vector1/1 -> Data Type Conversion1/1
  Data Type Conversion1/1 -> Multiport Switch/2
  Bus to Vector2/1 -> Data Type Conversion2/1
  Bus Selector2/1 -> Bus to Vector2/1
  Bus to Vector3/1 -> Data Type Conversion3/1
  Bus Selector3/1 -> Bus to Vector3/1
  Bus to Vector4/1 -> Data Type Conversion4/1
  Bus Selector4/1 -> Bus to Vector4/1
  Bus to Vector5/1 -> Data Type Conversion5/1
  Data Type Conversion5/1 -> Multiport Switch4/2
  Bus Selector5/1 -> Bus to Vector5/1
  Bus to Vector6/1 -> Data Type Conversion6/1
  Data Type Conversion6/1 -> Multiport Switch5/2
  Bus Selector6/1 -> Bus to Vector6/1
  Data Type Conversion4/1 -> Multiport Switch3/2
  Data Type Conversion3/1 -> Multiport Switch2/2
  Data Type Conversion2/1 -> Multiport Switch1/2
  Select_Signals/3(SW_DoorFR[Open0_1Closed]) -> Multiport Switch1/3
  Select_Signals/4(SW_DoorRL[Open0_1Closed]) -> Multiport Switch2/3
  Select_Signals/5(SW_DoorRR[Open0_1Closed]) -> Multiport Switch3/3
  Select_Signals/6(SW_Hood[Open0_1Closed]) -> Multiport Switch4/3
  Select_Signals/7(SW_Trunk[Open0_1Closed]) -> Multiport Switch5/3
  Multiport Switch4/1 -> Mux/5
  Multiport Switch5/1 -> Mux/6
  Multiport Switch3/1 -> Mux/4
  Multiport Switch2/1 -> Mux/3
  Multiport Switch1/1 -> Mux/2
  Multiport Switch/1 -> Mux/1
  Mux/1 -> Saturation/1
  Environment_Animation/1 -> Bus Selector2/1, Bus Selector6/1, Bus Selector5/1, Bus Selector4/1, Bus Selector3/1, Bus Selector1/1, Select_Signals/1(Fellow_Doors)
  Saturation/1 -> Fellow_Doors/1

== system ASM_AnimationInterface/AnimationInterface/Fellow_Lights ==
  Environment_Animation : Inport
  Bus Selector : BusSelector  OutputSignals=Fellow1_TurnLights,Fellow2_TurnLights,Fellow3_TurnLights,Fellow4_TurnLights,Fellow5_TurnLights,Fellow6_TurnLights,Fellow7_TurnLights,Fellow8_TurnLights,Fellow9_TurnLights,Fellow10_TurnLights,Fellow11_TurnLights,Fellow12_TurnLights,Fellow13_TurnLights,Fellow14_TurnLights,Fellow15_TurnLights,Fellow16_TurnLights,Fellow17_TurnLights,Fellow18_TurnLights,Fellow19_TurnLights,Fellow20_TurnLights,Fellow21_TurnLights,Fellow22_TurnLights,Fellow23_TurnLights,Fellow24_TurnLights,Fellow25_TurnLights,Fellow26_TurnLights,Fellow27_TurnLights,Fellow28_TurnLights,Fellow29_TurnLights,Fellow30_TurnLights  OutputAsBus=on
  Bus Selector2 : BusSelector  OutputSignals=a_Fellows[m|s2],Settings,UserSignals_Customized
  Bus to Vector3 : BusToVector
  Coding : Subsystem
  Compare_Both : simulink/Logic and Bit Operations/Compare To Constant  relop===  const=3  OutDataTypeStr=boolean
  Compare_Turnlight_L : simulink/Logic and Bit Operations/Compare To Constant  relop===  const=1  OutDataTypeStr=boolean
  Compare_Turnlight_R : simulink/Logic and Bit Operations/Compare To Constant  relop===  const=2  OutDataTypeStr=boolean
  Gain : Gain  Gain=-1
  Multiport Switch : MultiPortSwitch  Inputs=2  SaturateOnIntegerOverflow=off  InputSameDT=off
  Multiport Switch4 : MultiPortSwitch  Inputs=2  SaturateOnIntegerOverflow=off  InputSameDT=off
  Mux : Mux  Inputs=3
  OR : Logic  Operator=OR  IconShape=distinctive  AllPortsSameDT=off  OutDataTypeStr=boolean
  OR1 : Logic  Operator=OR  IconShape=distinctive  AllPortsSameDT=off  OutDataTypeStr=boolean
  Relay : Relay  OnSwitchValue=1.3  OffSwitchValue=1.2  OutDataTypeStr=boolean
  Select_Signals : Subsystem
  TurnLights[0|1|2|3] : DataTypeConversion  OutDataTypeStr=uint32  SaturateOnIntegerOverflow=off  RndMeth=Floor
  Fellow_Light : Outport  VectorParamsAs1DForOutWhenUnconnected=off
  wires:
  Bus Selector/1 -> Bus to Vector3/1
  Bus Selector2/3 -> Bus Selector/1  "<UserSignals_Customized>"
  Bus Selector2/1 -> Gain/1  "<a_Fellows[m|s2]>"
  Coding/1(Out) -> Fellow_Light/1
  TurnLights[0|1|2|3]/1 -> Multiport Switch4/2
  Relay/1 -> Multiport Switch/2
  Compare_Turnlight_L/1 -> OR/1
  Compare_Turnlight_R/1 -> OR1/1
  Multiport Switch/1 -> Mux/1
  Compare_Both/1 -> OR1/2, OR/2
  OR/1 -> Mux/2
  OR1/1 -> Mux/3
  Multiport Switch4/1 -> Compare_Turnlight_L/1, Compare_Turnlight_R/1, Compare_Both/1
  Mux/1 -> Coding/1(FellowLights)
  Bus to Vector3/1 -> TurnLights[0|1|2|3]/1
  Select_Signals/1(SW_ManualControl_Lights[1Scheduler|2Manual]) -> Multiport Switch4/1, Multiport Switch/1
  Select_Signals/2(SW_BrakeLight[0Off|1On]) -> Multiport Switch/3
  Select_Signals/3(SW_TurnLight[0Off|1Left|2Right|3Both]) -> Multiport Switch4/3
  Environment_Animation/1 -> Bus Selector2/1
  Bus Selector2/2 -> Select_Signals/1(Fellow_VehicleLights)  "<Settings>"
  Gain/1 -> Relay/1

== system ASM_AnimationInterface/AnimationInterface/OpenAnimationInterfaceModel ==

== system ASM_AnimationInterface/AnimationInterface/Vehicle_Doors ==
  Environment_Animation : Inport
  Bus Selector : BusSelector  OutputSignals=Mnv_DoorFL[],Mnv_DoorFR[],Mnv_DoorRL[],Mnv_DoorRR[],Mnv_Hood[],Mnv_Trunk[]  OutputAsBus=on
  Bus Selector7 : BusSelector  OutputSignals=Sw_ManualControl_Doors[1Maneuver|2Manual]
  Bus Selector8 : BusSelector  OutputSignals=Sw_DoorFL[0Closed_1Open],Sw_DoorFR[0Closed_1Open],Sw_DoorRL[0Closed_1Open],Sw_DoorRR[0Closed_1Open],Sw_Hood[0Closed_1Open],Sw_Trunk[0Closed_1Open]  OutputAsBus=on
  Bus to Vector : BusToVector
  Bus to Vector7 : BusToVector
  Data Type Conversion : DataTypeConversion  OutDataTypeStr=double  SaturateOnIntegerOverflow=off  RndMeth=Floor
  Data Type Conversion7 : DataTypeConversion  OutDataTypeStr=uint32  SaturateOnIntegerOverflow=off  RndMeth=Floor
  Data Type Conversion8 : DataTypeConversion  OutDataTypeStr=double  SaturateOnIntegerOverflow=off  RndMeth=Floor
  Multiport Switch6 : MultiPortSwitch  Inputs=2  OutMin=30  OutMax=30  OutDataTypeStr=double  SaturateOnIntegerOverflow=off
  Saturation : Saturate  UpperLimit=1  LowerLimit=0
  ASM_Vehicle_Doors : Outport  VectorParamsAs1DForOutWhenUnconnected=off
  wires:
  Bus Selector/1 -> Bus to Vector/1
  Environment_Animation/1 -> Bus Selector8/1, Bus Selector7/1, Bus Selector/1
  Data Type Conversion/1 -> Multiport Switch6/2
  Bus Selector8/1 -> Bus to Vector7/1
  Bus to Vector/1 -> Data Type Conversion/1
  Bus to Vector7/1 -> Data Type Conversion8/1
  Multiport Switch6/1 -> Saturation/1
  Data Type Conversion8/1 -> Multiport Switch6/3
  Bus Selector7/1 -> Data Type Conversion7/1  "<Sw_ManualControl_Doors[1Maneuver|2Manual]>"
  Data Type Conversion7/1 -> Multiport Switch6/1
  Saturation/1 -> ASM_Vehicle_Doors/1

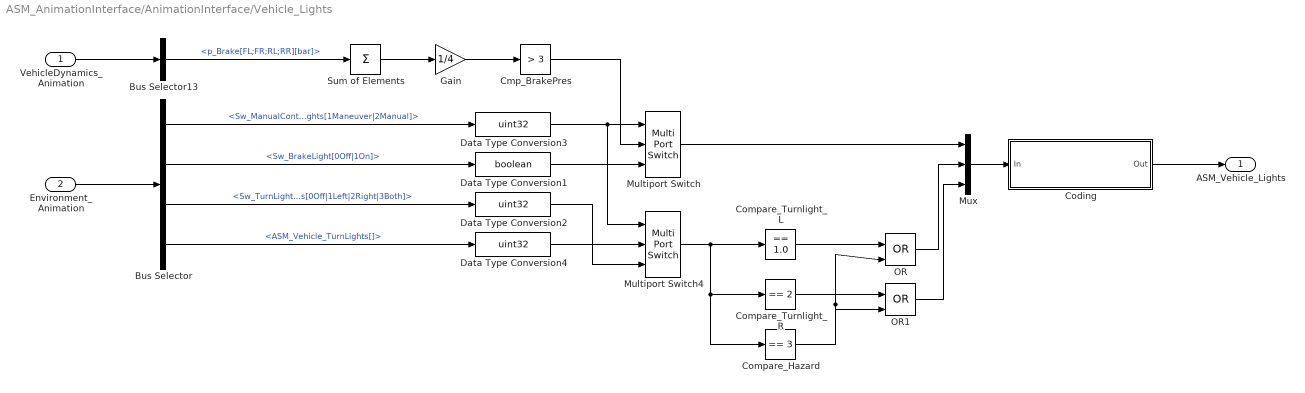
== system ASM_AnimationInterface/AnimationInterface/Vehicle_Lights ==
  VehicleDynamics_Animation : Inport
  Environment_Animation : Inport  Port=2
  Bus Selector : BusSelector  OutputSignals=Sw_ManualControl_Lights[1Maneuver|2Manual],Sw_BrakeLight[0Off|1On],Sw_TurnLights[0Off|1Left|2Right|3Both],ASM_Vehicle_TurnLights[]
  Bus Selector13 : BusSelector  OutputSignals=p_Brake[FL;FR;RL;RR][bar]
  Cmp_BrakePres : simulink/Logic and Bit Operations/Compare To Constant  relop=>  const=3  OutDataTypeStr=boolean
  Coding : Subsystem
  Compare_Hazard : simulink/Logic and Bit Operations/Compare To Constant  relop===  const=3  OutDataTypeStr=boolean
  Compare_Turnlight_L : simulink/Logic and Bit Operations/Compare To Constant  relop===  const=1.0  OutDataTypeStr=boolean
  Compare_Turnlight_R : simulink/Logic and Bit Operations/Compare To Constant  relop===  const=2  OutDataTypeStr=boolean
  Data Type Conversion1 : DataTypeConversion  OutDataTypeStr=boolean  SaturateOnIntegerOverflow=off  RndMeth=Floor
  Data Type Conversion2 : DataTypeConversion  OutDataTypeStr=uint32  SaturateOnIntegerOverflow=off  RndMeth=Floor
  Data Type Conversion3 : DataTypeConversion  OutDataTypeStr=uint32  SaturateOnIntegerOverflow=off  RndMeth=Floor
  Data Type Conversion4 : DataTypeConversion  OutDataTypeStr=uint32  SaturateOnIntegerOverflow=off  RndMeth=Floor
  Gain : Gain  Gain=1/4
  Multiport Switch : MultiPortSwitch  Inputs=2  SaturateOnIntegerOverflow=off  InputSameDT=off
  Multiport Switch4 : MultiPortSwitch  Inputs=2  SaturateOnIntegerOverflow=off  InputSameDT=off
  Mux : Mux  Inputs=3
  OR : Logic  Operator=OR  IconShape=distinctive  AllPortsSameDT=off  OutDataTypeStr=boolean
  OR1 : Logic  Operator=OR  IconShape=distinctive  AllPortsSameDT=off  OutDataTypeStr=boolean
  Sum of Elements : Sum  Inputs=+
  ASM_Vehicle_Lights : Outport  VectorParamsAs1DForOutWhenUnconnected=off
  wires:
  VehicleDynamics_Animation/1 -> Bus Selector13/1
  Environment_Animation/1 -> Bus Selector/1
  Coding/1(Out) -> ASM_Vehicle_Lights/1
  Mux/1 -> Coding/1(In)
  Multiport Switch4/1 -> Compare_Turnlight_L/1, Compare_Turnlight_R/1, Compare_Hazard/1
  Data Type Conversion1/1 -> Multiport Switch/3
  OR/1 -> Mux/2
  Data Type Conversion2/1 -> Multiport Switch4/3
  Cmp_BrakePres/1 -> Multiport Switch/2
  OR1/1 -> Mux/3
  Compare_Turnlight_R/1 -> OR1/1
  Bus Selector/2 -> Data Type Conversion1/1  "<Sw_BrakeLight[0Off|1On]>"
  Bus Selector/4 -> Data Type Conversion4/1  "<ASM_Vehicle_TurnLights[]>"
  Sum of Elements/1 -> Gain/1
  Data Type Conversion4/1 -> Multiport Switch4/2
  Bus Selector/3 -> Data Type Conversion2/1  "<Sw_TurnLights[0Off|1Left|2Right|3Both]>"
  Bus Selector/1 -> Data Type Conversion3/1  "<Sw_ManualControl_Lights[1Maneuver|2Manual]>"
  Compare_Hazard/1 -> OR1/2, OR/2
  Data Type Conversion3/1 -> Multiport Switch4/1, Multiport Switch/1
  Multiport Switch/1 -> Mux/1
  Gain/1 -> Cmp_BrakePres/1
  Compare_Turnlight_L/1 -> OR/1
  Bus Selector13/1 -> Sum of Elements/1  "<p_Brake[FL;FR;RL;RR][bar]>"
